simulink model "grid_following_dqctrl_delta"  (R2026b)
settings: Solver=VariableStepAuto
undefined symbols (not defined in the file or in its folder): param
libraries: nesl_utility x2, grid_following_dqctrl x1, afe_ssc_lib x1
settings Model: Creator=d.bagnara  LastModifiedBy=d.bagnara

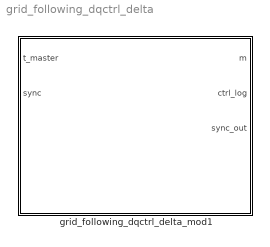
== system grid_following_dqctrl_delta ==
  grid_following_dqctrl_delta_mod1 : Subsystem  mask(Grid-following AFE (two-level bridge, LCL filter, delta capacitors)){p=param.afe_follower(1)}
      mask prompts: p "Parameter struct p (afe_follower_module_param)"
      mask help: Grid-following AFE (DC-link voltage control, FHT-PLL) in one block with the filter capacitors in DELTA: grid_following_dqctrl with the Simscape component afe_ssc.afe_two_level_lcl_delta (ideal two-level bridge, DC-link capacitor, LCL filter with delta capacitors) as power stage. Same ports, mask parameter p, control and Help as grid_following_dqctrl, so the two blocks can be swapped. p.hw.Cf and p.hw.Rcf keep their meaning in grid_following_dqctrl (per-phase values of the star): the block puts p.hw.Cf/3 and 3*p.hw.Rcf in each delta branch, so the same p gives the same filter and the same control behaviour. Control and PWM: library link to the MATLAB Function afe_dq_follower_ctrl_pwm of grid_following_dqctrl (afe_follower_ctrl_pwm): a change of the control code there applies to this block too. Measurements to the control through a Unit Delay of one tc. Ports: ug_a/b/c left, Udc(+)/Udc(-) right, t_master and sync in, m (17x1 pu), ctrl_log (45x1) and sync_out out (master/slave as in grid_following_dqctrl: p.ctrl.slave = 1 takes the current references of the master from sync). m(1:14) as in grid_following_dqctrl (m(4:6) = capacitor node voltages without zero sequence, the voltages of the equivalent star); m(15:17) = currents of the three delta capacitors [icf_ab; icf_bc; icf_ca] in pu of ibez, icf_ab from node a to node b; the current from line a into the capacitors is m(15) - m(17). Parameter p: struct with the fields hw, pwm, ctrl, e.g. grid_following_param_example.m of this folder. Made by tools/make_dqctrl_delta.py from grid_following_dqctrl.slx. Description and user guide: the Help of this block (note library/documentation/grid_forming_following_afe).
      mask Help: eval('pwrdoc = which(''grid_forming_following_afe.pdf''); if isempty(pwrdoc), pwrdoc = ''https://github.com/pwr-control/library/blob/main/library/documentation/grid_forming_following_afe/grid_forming_following_afe.pdf''; end; web(pwrdoc, ''-browser''); clear pwrdoc')
      mask Display:
      | port_label('LConn', 1, 'ug_a');
      | port_label('LConn', 2, 'ug_b');
      | port_label('LConn', 3, 'ug_c');
      | port_label('RConn', 1, 'Udc(+)');
      | port_label('RConn', 2, 'Udc(-)');
      | port_label('input', 1, 't_master');
      | port_label('input', 2, 'sync');
      | port_label('output', 1, 'M');
      | port_label('output', 2, 'ctrl_log');
      | port_label('output', 3, 'sync_out');

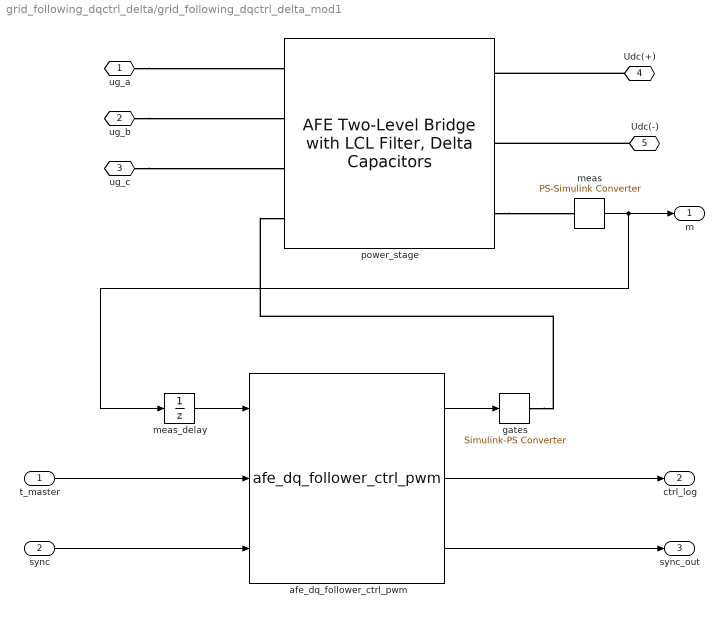
== system grid_following_dqctrl_delta/grid_following_dqctrl_delta_mod1 ==
  t_master : Inport
  sync : Inport  Port=2
  afe_dq_follower_ctrl_pwm : grid_following_dqctrl/grid_following_dqctrl_mod1/afe_dq_follower_ctrl_pwm  SystemSampleTime=-1  VariantActivationTime=update diagram  EmptyChoice=off  PassThrough=off  PassThroughVariantControl=(default)  EmptyChoiceVariantControl=(default)  AllowFlexibleInterface=on  Latency=0  AutoFrameSizeCalculation=off
  gates : nesl_utility/Simulink-PS Converter  PhysicalDomain=network_engine_domain  SubClassName=ps_input  LeftPortType=input  RightPortType=output  PseudoPeriodic=off  Frequencies=[]  NoiseDistribution=none  NoiseParameters=[]  Unit=V  AffineConversion=off  FilteringAndDerivatives=provide  SimscapeFilterOrder=1  InputFilterTimeConstant=0.001  UdotUserProvided=0
  meas : nesl_utility/PS-Simulink Converter  PhysicalDomain=network_engine_domain  SubClassName=ps_output  LeftPortType=input  RightPortType=output  PseudoPeriodic=off  Frequencies=[]  VectorFormat=inherit  Unit=1  AffineConversion=off
  meas_delay : UnitDelay  SampleTime=p.pwm.tc
  power_stage : afe_ssc_lib/AFE Two-Level Bridge with LCL Filter, Delta Capacitors  Vth=p.hw.Vth V  Ron=p.hw.Ron Ohm  Goff=p.hw.Goff 1/Ohm  cap_dc=afe_ssc.onoff.on  Cdc=p.hw.Cdc F  Rdc=p.hw.Rdc Ohm  L1p=p.hw.L1p H  L10=p.hw.L10 H  R1=p.hw.R1 Ohm  Lls1=p.hw.Lls1 H  Cf=p.hw.Cf/3 F  Rcf=3*p.hw.Rcf Ohm  L2p=p.hw.L2p H  L20=p.hw.L20 H  R2=p.hw.R2 Ohm  Lls2=p.hw.Lls2 H  ubez=p.hw.ubez V  ibez=p.hw.ibez A  udc_nom=p.hw.udc_nom V  vdc_specify=off  vdc_priority=None  vdc=0 V  vdc_nominal_specify=off  vdc_nominal_value=1  vdc_nominal_unit=V  vcap_specify=off  vcap_priority=None  vcap=0 V  vcap_nominal_specify=off  vcap_nominal_value=1  vcap_nominal_unit=V  ic_specify=off  ic_priority=None  ic=0 A  ic_nominal_specify=off  ic_nominal_value=1  ic_nominal_unit=A  vm_a_specify=off  vm_a_priority=None  vm_a=0 V  vm_a_nominal_specify=off  vm_a_nominal_value=1  vm_a_nominal_unit=V  vm_b_specify=off  vm_b_priority=None  vm_b=0 V  vm_b_nominal_specify=off  vm_b_nominal_value=1  vm_b_nominal_unit=V  vm_c_specify=off  vm_c_priority=None  vm_c=0 V  vm_c_nominal_specify=off  vm_c_nominal_value=1  vm_c_nominal_unit=V  i_ah_specify=off  i_ah_priority=None  i_ah=0 A  i_ah_nominal_specify=off  i_ah_nominal_value=1  i_ah_nominal_unit=A  i_al_specify=off  i_al_priority=None  i_al=0 A  i_al_nominal_specify=off  i_al_nominal_value=1  i_al_nominal_unit=A  i_bh_specify=off  i_bh_priority=None  i_bh=0 A  i_bh_nominal_specify=off  i_bh_nominal_value=1  i_bh_nominal_unit=A  i_bl_specify=off  i_bl_priority=None  i_bl=0 A  i_bl_nominal_specify=off  i_bl_nominal_value=1  i_bl_nominal_unit=A  i_ch_specify=off  i_ch_priority=None  i_ch=0 A  i_ch_nominal_specify=off  i_ch_nominal_value=1  i_ch_nominal_unit=A  i_cl_specify=off  i_cl_priority=None  i_cl=0 A  i_cl_nominal_specify=off  i_cl_nominal_value=1  i_cl_nominal_unit=A  i1_a_specify=off  i1_a_priority=None  i1_a=0 A  i1_a_nominal_specify=off  i1_a_nominal_value=1  i1_a_nominal_unit=A  i1_b_specify=off  i1_b_priority=None  i1_b=0 A  i1_b_nominal_specify=off  i1_b_nominal_value=1  i1_b_nominal_unit=A  i1_c_specify=off  i1_c_priority=None  i1_c=0 A  i1_c_nominal_specify=off  i1_c_nominal_value=1  i1_c_nominal_unit=A  vk_a_specify=off  vk_a_priority=None  vk_a=0 V  vk_a_nominal_specify=off  vk_a_nominal_value=1  vk_a_nominal_unit=V  vk_b_specify=off  vk_b_priority=None  vk_b=0 V  vk_b_nominal_specify=off  vk_b_nominal_value=1  vk_b_nominal_unit=V  vk_c_specify=off  vk_c_priority=None  vk_c=0 V  vk_c_nominal_specify=off  vk_c_nominal_value=1  vk_c_nominal_unit=V  vc_ab_specify=off  vc_ab_priority=None  vc_ab=0 V  vc_ab_nominal_specify=off  vc_ab_nominal_value=1  vc_ab_nominal_unit=V  vc_bc_specify=off  vc_bc_priority=None  vc_bc=0 V  vc_bc_nominal_specify=off  vc_bc_nominal_value=1  vc_bc_nominal_unit=V  vc_ca_specify=off  vc_ca_priority=None  vc_ca=0 V  vc_ca_nominal_specify=off  vc_ca_nominal_value=1  vc_ca_nominal_unit=V  icf_ab_specify=off  icf_ab_priority=None  icf_ab=0 A  icf_ab_nominal_specify=off  icf_ab_nominal_value=1  icf_ab_nominal_unit=A  icf_bc_specify=off  icf_bc_priority=None  icf_bc=0 A  icf_bc_nominal_specify=off  icf_bc_nominal_value=1  icf_bc_nominal_unit=A  icf_ca_specify=off  icf_ca_priority=None  icf_ca=0 A  icf_ca_nominal_specify=off  icf_ca_nominal_value=1  icf_ca_nominal_unit=A  i2_a_specify=off  i2_a_priority=None  i2_a=0 A  i2_a_nominal_specify=off  i2_a_nominal_value=1  i2_a_nominal_unit=A  i2_b_specify=off  i2_b_priority=None  i2_b=0 A  i2_b_nominal_specify=off  i2_b_nominal_value=1  i2_b_nominal_unit=A  i2_c_specify=off  i2_c_priority=None  i2_c=0 A  i2_c_nominal_specify=off  i2_c_nominal_value=1  i2_c_nominal_unit=A
  ug_a : PMIOPort  Side=Left
  ug_b : PMIOPort  Port=2  Side=Left
  ug_c : PMIOPort  Port=3  Side=Left
  Udc(+) : PMIOPort  Port=4  Side=Right
  Udc(-) : PMIOPort  Port=5  Side=Right
  m : Outport
  ctrl_log : Outport  Port=2
  sync_out : Outport  Port=3
  wires:
  t_master/1 -> afe_dq_follower_ctrl_pwm/2
  meas/1 -> m/1, meas_delay/1
  meas_delay/1 -> afe_dq_follower_ctrl_pwm/1
  afe_dq_follower_ctrl_pwm/1 -> gates/1
  afe_dq_follower_ctrl_pwm/2 -> ctrl_log/1
  sync/1 -> afe_dq_follower_ctrl_pwm/3
  afe_dq_follower_ctrl_pwm/3 -> sync_out/1
  connections:
  gates/RConn1 -- power_stage/LConn4
  power_stage/RConn3 -- meas/LConn1
  ug_a/RConn1 -- power_stage/LConn1
  ug_b/RConn1 -- power_stage/LConn2
  ug_c/RConn1 -- power_stage/LConn3
  Udc(+)/RConn1 -- power_stage/RConn1
  Udc(-)/RConn1 -- power_stage/RConn2
